simulink model "ps5_stage05_pi_hardware_matched_R2024a"  (R2024a)
settings: Solver=FixedStepDiscrete  StartTime=0.0  StopTime=10  FixedStep=0.002  RelTol=1e-3
libraries: slpidlib x1
settings Model: Creator=tanuj  LastModifiedBy=tanuj

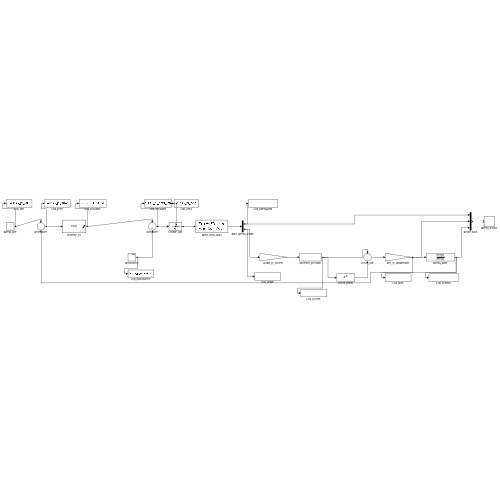
[thumbnail: Simulink's stored preview of the top-level diagram]
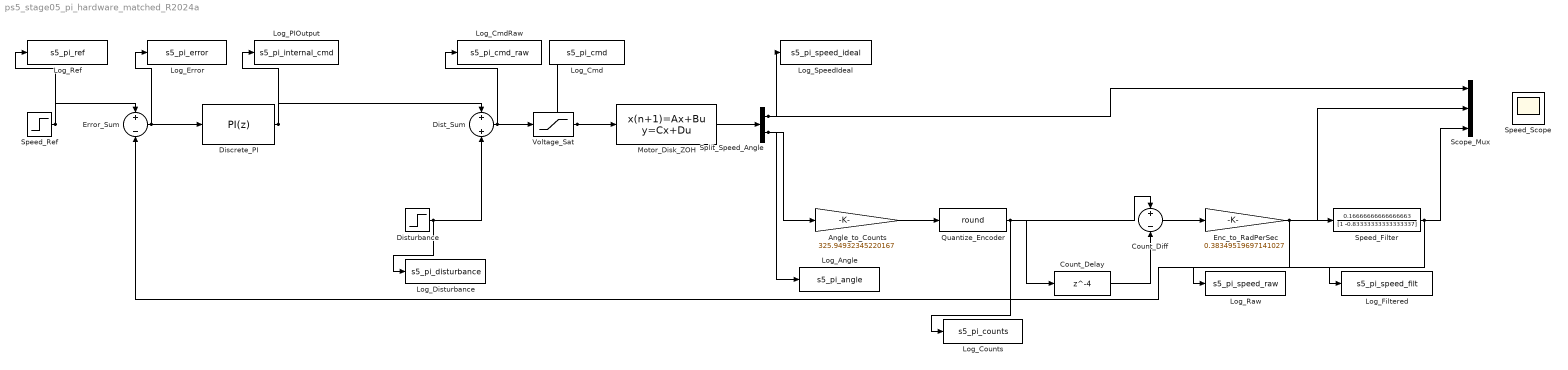
== system ps5_stage05_pi_hardware_matched_R2024a ==
  Angle_to_Counts : Gain  Gain=325.94932345220167
  Count_Delay : Delay  DelayLength=4  InitialCondition=0  SampleTime=0.002
  Count_Diff : Sum  Inputs=+-
  Discrete_PI : slpidlib/PID Controller  Controller=PI  Form=Parallel  TimeDomain=Discrete-time  UseExternalTs=off  SampleTime=0.002  IntegratorMethod=Forward Euler  FilterMethod=Forward Euler  ControllerParametersSource=internal  P=0.1659645524035018  I=5.2040475778402975  UseKiTs=off  D=0  UseExternalDerivativeSource=off  N=100  UseFilter=on  TunerSelectOption=Transfer Function Based (PID Tuner App)  InitialConditionSource=internal  InitialConditionForIntegrator=0  InitialConditionForFilter=0  DifferentiatorICPrevScaledInput=0  ExternalReset=none  TrackingMode=off  Kt=1  LimitOutput=on  SatLimitsSource=internal  UpperSaturationLimit=10  LowerSaturationLimit=-10  LinearizeAsGain=on  AntiWindupMode=clamping  Kb=1  LimitIntegrator=off  UpperIntegratorSaturationLimit=inf  LowerIntegratorSaturationLimit=-inf  POutMin=[]  POutMax=[]  IOutMin=[]  IOutMax=[]  DOutMin=[]  DOutMax=[]  NOutMin=[]  NOutMax=[]  SumOutMin=[]  SumOutMax=[]  SaturationOutMin=[]  SaturationOutMax=[]  PParamMin=[]  PParamMax=[]  IParamMin=[]  IParamMax=[]  DParamMin=[]  DParamMax=[]  NParamMin=[]  NParamMax=[]  KbParamMin=[]  KbParamMax=[]  KtParamMin=[]  KtParamMax=[]  KbOutMin=[]  KbOutMax=[]  KtOutMin=[]  KtOutMax=[]  IntegratorOutMin=[]  IntegratorOutMax=[]  FilterOutMin=[]  FilterOutMax=[]  SumI1OutMin=[]  SumI1OutMax=[]  SumI2OutMin=[]  SumI2OutMax=[]  SumI3OutMin=[]  SumI3OutMax=[]  SumI4OutMin=[]  SumI4OutMax=[]  SumDOutMin=[]  SumDOutMax=[]  DifferentiatorOutMin=[]  DifferentiatorOutMax=[]  FilterDiffOutCoefMin=[]  FilterDiffOutCoefMax=[]  ReciprocalOutMin=[]  ReciprocalOutMax=[]  SumDenOutMin=[]  SumDenOutMax=[]  SumNumOutMin=[]  SumNumOutMax=[]  DivideOutMin=[]  DivideOutMax=[]  UdiffTsProdOutMin=[]  UdiffTsProdOutMax=[]  NTsProdOutMin=[]  NTsProdOutMax=[]  UintegralTsProdOutMin=[]  UintegralTsProdOutMax=[]  UngainTsProdOutMin=[]  UngainTsProdOutMax=[]  ClampingZeroOutDataTypeStr=Inherit: Inherit via back propagation  ClampingZeroOutMin=[]  ClampingZeroOutMax=[]  FilterDenConstantOutDataTypeStr=Inherit: Inherit via back propagation  FilterDenConstantOutMin=[]  FilterDenConstantOutMax=[]  PCopyOutDataTypeStr=Inherit: Inherit via back propagation  PCopyOutMin=[]  PCopyOutMax=[]  NCopyOutDataTypeStr=Inherit: Inherit via back propagation  NCopyOutMin=[]  NCopyOutMax=[]  IntegratorContinuousStateAttributes=''  IntegratorStateMustResolveToSignalObject=off  IntegratorRTWStateStorageClass=Auto  FilterContinuousStateAttributes=''  FilterStateMustResolveToSignalObject=off  FilterRTWStateStorageClass=Auto  ParallelPVariant=InternalParameters  IdealPVariant=Disabled  IVariant=InternalParameters  DVariant=Disabled  IntegratorVariant=Discrete  SatVariant=Enabled  AWVariant=DiscClampingParallel  PCopyVariant=Disabled  TRVariant=Disabled  FdbkBlocksVariant=Forward  IdealPFdbkVariant=Disabled  SatFdbkVariant=Disabled  DerivativeFilterVariant=Disabled  NVariant=Disabled  NCopyVariant=Disabled_SignalSpec  FilterICVariant=Disabled  IntegratorICVariant=InternalICs  ExternalResetVariant=Disabled  TRSumVariant=Passthrough  SumFdbkVariant=Disabled  SumVariant=Sum_PI  TsampFilterVariant=InternalTs  TsampNgainVariant=Passthrough  TsampIntegralVariant=Disabled_SignalSpec  ExternalSaturationOutDataTypeStr=Inherit: Same as second input  DerivativeSourceVariant=Disabled
  Dist_Sum : Sum
  Disturbance : Step  Time=5  After=0.5  SampleTime=0.002
  Enc_to_RadPerSec : Gain  Gain=0.38349519697141027
  Error_Sum : Sum  Inputs=+-
  Log_Angle : ToWorkspace  VariableName=s5_pi_angle  SampleTime=-1
  Log_Cmd : ToWorkspace  VariableName=s5_pi_cmd  SampleTime=-1
  Log_CmdRaw : ToWorkspace  VariableName=s5_pi_cmd_raw  SampleTime=-1
  Log_Counts : ToWorkspace  VariableName=s5_pi_counts  SampleTime=-1
  Log_Disturbance : ToWorkspace  VariableName=s5_pi_disturbance  SampleTime=-1
  Log_Error : ToWorkspace  VariableName=s5_pi_error  SampleTime=-1
  Log_Filtered : ToWorkspace  VariableName=s5_pi_speed_filt  SampleTime=-1
  Log_PIOutput : ToWorkspace  VariableName=s5_pi_internal_cmd  SampleTime=-1
  Log_Raw : ToWorkspace  VariableName=s5_pi_speed_raw  SampleTime=-1
  Log_Ref : ToWorkspace  VariableName=s5_pi_ref  SampleTime=-1
  Log_SpeedIdeal : ToWorkspace  VariableName=s5_pi_speed_ideal  SampleTime=-1
  Motor_Disk_ZOH : DiscreteStateSpace  A=[-0.0019480304943638347 -0.0055041701060564701 0;0.34591769089835145 0.9762812537573784 0;0.00064636393789134212 0.0019778638926502613 1]  B=[0.13043057123356561;0.56205559816638462;0.00052455230686583696]  C=[0 1 0;0 0 1]  D=[0;0]  SampleTime=0.002
  Quantize_Encoder : Rounding  Operator=round
  Scope_Mux : Mux  Inputs=3
  Speed_Filter : DiscreteFilter  Numerator=0.16666666666666663  Denominator=[1 -0.83333333333333337]  SampleTime=0.002
  Speed_Ref : Step  After=50  SampleTime=0.002
  Speed_Scope : Scope
  Split_Speed_Angle : Demux  Outputs=2
  Voltage_Sat : Saturate  UpperLimit=10  LowerLimit=-10
  wires:
  Speed_Ref/1 -> Error_Sum/1, Log_Ref/1
  Error_Sum/1 -> Discrete_PI/1, Log_Error/1
  Discrete_PI/1 -> Dist_Sum/1, Log_PIOutput/1
  Disturbance/1 -> Dist_Sum/2, Log_Disturbance/1
  Dist_Sum/1 -> Voltage_Sat/1, Log_CmdRaw/1
  Voltage_Sat/1 -> Motor_Disk_ZOH/1, Log_Cmd/1
  Motor_Disk_ZOH/1 -> Split_Speed_Angle/1
  Split_Speed_Angle/2 -> Angle_to_Counts/1, Log_Angle/1
  Angle_to_Counts/1 -> Quantize_Encoder/1
  Quantize_Encoder/1 -> Count_Diff/1, Count_Delay/1, Log_Counts/1
  Count_Delay/1 -> Count_Diff/2
  Count_Diff/1 -> Enc_to_RadPerSec/1
  Enc_to_RadPerSec/1 -> Speed_Filter/1, Log_Raw/1, Scope_Mux/2
  Speed_Filter/1 -> Error_Sum/2, Log_Filtered/1, Scope_Mux/3
  Split_Speed_Angle/1 -> Log_SpeedIdeal/1, Scope_Mux/1
